simulink model "untitled"  (R2020a)
settings: Solver=VariableStepAuto  StartTime=0.0  StopTime=100  RelTol=1e-3
libraries: fl_lib x4, nesl_utility x4, ee_lib x3
settings Model: Creator=Win10  LastModifiedBy=Win10

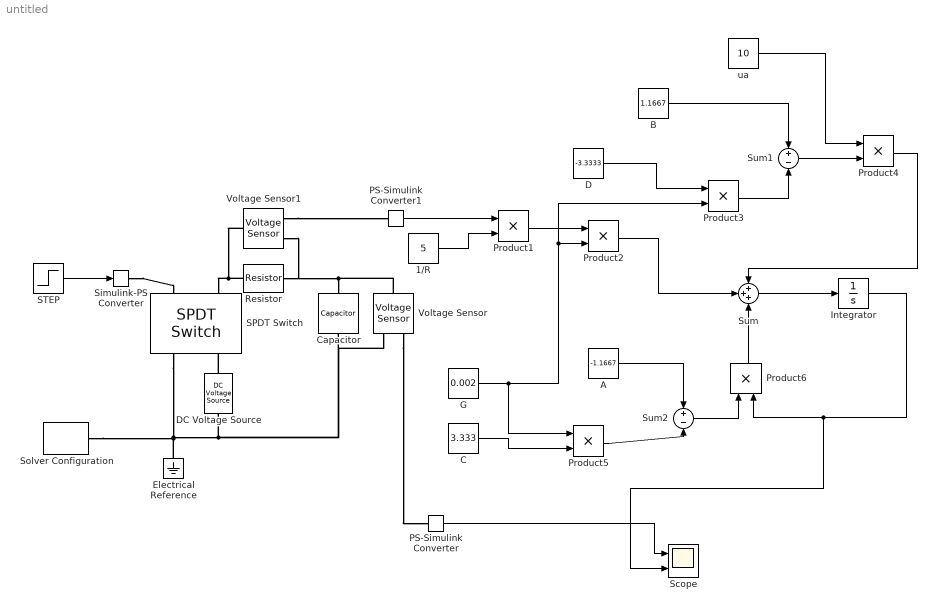
== system untitled ==
  1/R : Constant  Value=5
  A : Constant  Value=-1.1667
  B : Constant  Value=1.1667
  C : Constant  Value=3.333
  Capacitor : ee_lib/Passive/Capacitor  cap_option=0  c=2.85714 F  Cvec=[1e-05, 1e-06] F  Vvec=[0, 10] V  CV_table_symmetry=1  f_vec=[1, 10] kHz  DFext_vec=[.8, 1.2]  C_tol=5  enable_C_tol=0  tol_distribution=1  nSigma=4  r=0 Ohm  g=0 1/Ohm  averaging_period=0 s  enable_operating_limits=0  operating_limit_action=2  max_working_voltage_range=[-25, 25] V  power_rating=1 W  enable_faults=0  fault_action=1  Cscale_faulted=100  R_faulted=1e-3 Ohm  G_faulted=0 1/Ohm  tau_fault=1e-3 s  enable_temporal_fault=0  t_fault=1 s  enable_behavioral_fault=0  max_permissible_voltage_range=[-100, 100] V  t_fail_on_voltage=1 s  i_specify=off  i_priority=None  i=0 A  i_nominal_specify=off  i_nominal_unit=A  i_nominal_value=1  v_specify=off  v_priority=None  v=0 V  v_nominal_specify=off  v_nominal_unit=V  v_nominal_value=1  vc_specify=off  vc_priority=High  vc=0 V  vc_nominal_specify=off  vc_nominal_unit=V  vc_nominal_value=1
  D : Constant  Value=-3.3333
  DC Voltage Source : fl_lib/Electrical/Electrical Sources/DC Voltage Source  v0=10 V
  Electrical Reference : fl_lib/Electrical/Electrical Elements/Electrical Reference
  G : Constant  Value=0.002
  Integrator : Integrator
  PS-Simulink Converter : nesl_utility/PS-Simulink Converter  PhysicalDomain=network_engine_domain  SubClassName=ps_output  LeftPortType=input  RightPortType=output  PseudoPeriodic=off  Frequencies=[]  Unit=inherit  AffineConversion=off
  PS-Simulink Converter1 : nesl_utility/PS-Simulink Converter  PhysicalDomain=network_engine_domain  SubClassName=ps_output  LeftPortType=input  RightPortType=output  PseudoPeriodic=off  Frequencies=[]  Unit=inherit  AffineConversion=off
  Product{1..6} (6 alike) : Product
  Resistor : ee_lib/Passive/Resistor  R=0.2 Ohm  R_tol=5  enable_R_tol=0  tol_distribution=1  nSigma=4  enable_operating_limits=0  operating_limit_action=2  max_working_voltage=100 V  power_rating=1 W  enable_faults=0  fault_action=1  R_faulted=inf Ohm  enable_temporal_fault=0  t_fault=1 s  enable_behavioral_fault=0  max_permissible_current=1 A  t_fail_on_current=1 s  noise_mode=0  sample_time=1e-3 s  repeatability=1  auto_seed=418932850  user_seed=0  Tdevice=25 degC  alpha=3.93e-3 1/K  Tmeas=25 degC  thermal_mass=100 J/K  power_derating_T1=70 degC  power_derating_T2=155 degC  operating_temperature_range_vec=[-50, 150] degC  temperature_specify=off  temperature_priority=High  temperature=298.15 K  temperature_nominal_specify=off  temperature_nominal_unit=K  temperature_nominal_value=1
  SPDT Switch : ee_lib/Switches & Breakers/SPDT Switch  R_closed=0.01 Ohm  G_open=1e-6 S  Threshold=0.5 V  Width=0 V  model_dynamics=0  t_on=1e-3 s  t_off=1e-3 s  initial_vT=0 V
      settings: SourceProductBaseCode=PS
  STEP : Step  SampleTime=0
  Scope : Scope  NumInputPorts=2
  "Simulink-PS Converter " : nesl_utility/Simulink-PS Converter  PhysicalDomain=network_engine_domain  SubClassName=ps_input  LeftPortType=input  RightPortType=output  PseudoPeriodic=off  Frequencies=[]  NoiseDistribution=none  NoiseParameters=[]  Unit=1  AffineConversion=off  FilteringAndDerivatives=provide  SimscapeFilterOrder=1  InputFilterTimeConstant=0.001  UdotUserProvided=0
  Solver Configuration : nesl_utility/Solver Configuration  PhysicalDomain=network_engine_domain  SubClassName=solver  LeftPortType=input  RightPortType=generic  Tones=[]  Harmonics=[]  SimulateNoise=off  Profile=off  UseLocalSampling=off  EnableSwitchedLinearOptims=on  FrequencyDomain=off  UseCCode=off  RelTol=0.001  AbsTol=1e-06  MinStep=1e-09  ToWorkspace=off  RevertToSquareIcSolve=off  NumHomotopyIterations=100  PhasorMode=off  PhasorModeNumHarmonics=1  DoDC=off  ResidualTolerance=1e-09  UseLocalSolver=off  LocalSolverChoice=NE_BACKWARD_EULER_ADVANCER  LocalSolverSampleTime=0.001  DoFixedCost=off  MaxNonlinIter=3  MaxModeIter=2  LinearAlgebra=auto  EquationFormulation=NE_TIME_EF  DelaysMemoryBudget=1024  AutomaticFiltering=on  FilteringTimeConstant=0.001  PartitionStorageMethod=AS_NEEDED  PartitionMemoryBudget=1024  PartitionMethod=ROBUST
  Sum : Sum  Inputs=+++
  Sum1 : Sum  Inputs=+|-
  Sum2 : Sum  Inputs=+|-
  Voltage Sensor : fl_lib/Electrical/Electrical Sensors/Voltage Sensor
  Voltage Sensor1 : fl_lib/Electrical/Electrical Sensors/Voltage Sensor
  ua : Constant  Value=10
  wires:
  STEP/1 -> "Simulink-PS Converter "/1
  PS-Simulink Converter/1 -> Scope/1
  PS-Simulink Converter1/1 -> Product1/1
  1/R/1 -> Product1/2
  Product1/1 -> Product2/1
  G/1 -> Product3/2, Product2/2, Product5/1
  Product2/1 -> Sum/2
  B/1 -> Sum1/1
  Product3/1 -> Sum1/2
  D/1 -> Product3/1
  Sum1/1 -> Product4/2
  Product4/1 -> Sum/1
  C/1 -> Product5/2
  A/1 -> Sum2/1
  Product5/1 -> Sum2/2
  Sum/1 -> Integrator/1
  Product6/1 -> Sum/3
  Sum2/1 -> Product6/1
  ua/1 -> Product4/1
  Integrator/1 -> Scope/2, Product6/2
  connections:
  Capacitor/LConn1 -- Voltage Sensor1/RConn2 -- Resistor/RConn1 -- Voltage Sensor/LConn1
  Electrical Reference/LConn1 -- Voltage Sensor/RConn2 -- Capacitor/RConn1 -- DC Voltage Source/RConn1 -- SPDT Switch/RConn1 -- Solver Configuration/RConn1
  Resistor/LConn1 -- Voltage Sensor1/LConn1 -- SPDT Switch/LConn2
  Voltage Sensor/RConn1 -- PS-Simulink Converter/LConn1
  DC Voltage Source/LConn1 -- SPDT Switch/RConn2
  "Simulink-PS Converter "/RConn1 -- SPDT Switch/LConn1
  Voltage Sensor1/RConn1 -- PS-Simulink Converter1/LConn1
